simulink library "acc_control_lib"  (R2024a)
settings: Solver=VariableStepAuto  StartTime=0.0  StopTime=10.0  RelTol=1e-3
settings Model: Creator=26401  LastModifiedBy=26401

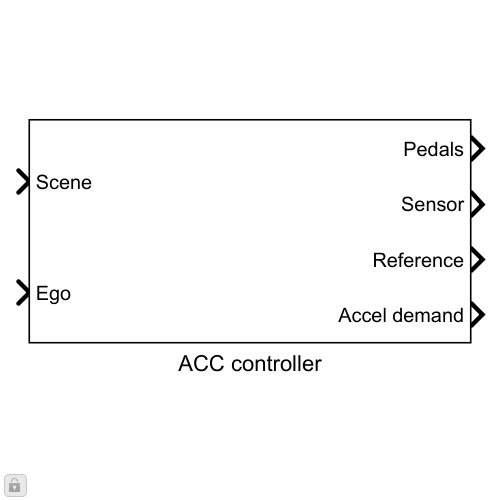
[thumbnail: Simulink's stored preview of the top-level diagram]
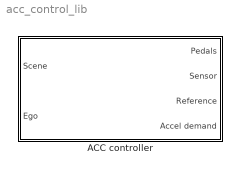
== system acc_control_lib ==
  ACC controller : Subsystem

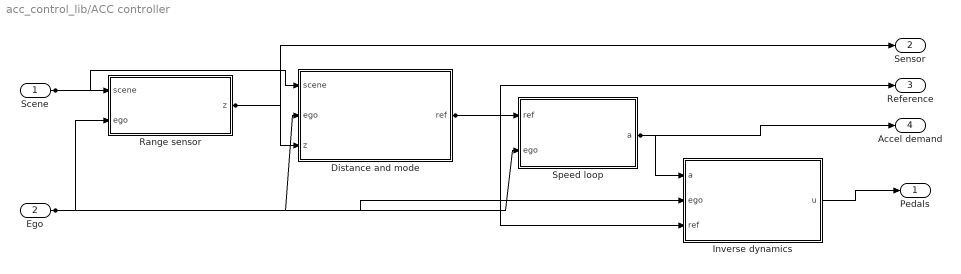
== system acc_control_lib/ACC controller ==
  Scene : Inport
  Ego : Inport  Port=2
  Distance and mode : MATLAB Function  TreatAsAtomicUnit=on
  Inverse dynamics : MATLAB Function  TreatAsAtomicUnit=on
  Range sensor : MATLAB Function  TreatAsAtomicUnit=on
  Speed loop : MATLAB Function  TreatAsAtomicUnit=on
  Pedals : Outport
  Sensor : Outport  Port=2
  Reference : Outport  Port=3
  Accel demand : Outport  Port=4
  wires:
  Scene/1 -> Range sensor/1(scene), Distance and mode/1(scene)
  Ego/1 -> Range sensor/2(ego), Distance and mode/2(ego), Speed loop/2(ego), Inverse dynamics/2(ego)
  Range sensor/1(z) -> Distance and mode/3(z), Sensor/1
  Distance and mode/1(ref) -> Speed loop/1(ref), Inverse dynamics/3(ref), Reference/1
  Speed loop/1(a) -> Inverse dynamics/1(a), Accel demand/1
  Inverse dynamics/1(u) -> Pedals/1

== matlab function acc_control_lib/ACC controller/Range sensor ==
  data: scene input; z output; ego input
function z = range_sensor(scene,ego)
% scene = [set speed, lead speed, lead rear s, target exists].
% ego = [front bumper s, speed, acceleration, engine rpm, transmission ratio].
% Negative gap remains visible for collision detection in a single-lane run.
gap = scene(3)-ego(1);
valid = scene(4)>0.5 && gap<=150;
z = [double(valid);0;0];
if valid
    z(2:3) = [gap;scene(2)-ego(2)];
end
end

== matlab function acc_control_lib/ACC controller/Speed loop ==
  data: ref input; a output; ego input
function a = speed_control(ref,ego)
% Inner P speed feedback, no integral accumulation across mode transitions.
% Local gains and slew limits. Requests refer to net longitudinal acceleration.
persistent previous
if isempty(previous)
    previous = 0;
end
demand = min(max(2.4*(ref(1)-ego(2)),-4),2.8);
if ref(4)>0.5
    demand = -1.0;
end
a = previous + min(max(demand-previous,-6*0.02),6*0.02);
previous = a;
end

== matlab function acc_control_lib/ACC controller/Inverse dynamics ==
  data: a input; u output; ego input; ref input
function u = inverse_actuators(a,ego,ref)
% Drive/brake hysteresis around the zero-pedal coasting acceleration.
% Throttle is normalized, master-cylinder pressure is in MPa.
persistent driving
if isempty(driving)
    driving = true;
end
[loss,fullForce,mass] = baseline_forces(ego(2),ego(4),ego(5));
coast = -loss/mass;
if a>coast+0.05
    driving = true;
elseif a<coast-0.05
    driving = false;
end
force = mass*(a-coast);
throttle = 0;
pressure = 0;
if driving
    throttle = min(max(force/fullForce,0),1);
else
    torque = max(-force*0.304,0);
    % Two front (350 N m/MPa) and two rear (200 N m/MPa) brakes.
    % Above 2 MPa the rear pressure slope falls to 0.3.
    if torque <= 2200
        pressure = torque/1100;
    else
        pressure = 2+(torque-2200)/820;
    end
    pressure = min(pressure,8);
end
if ref(4)>0.5
    throttle = 0; pressure = max(pressure,0.6); driving = false;
end
u = [throttle;pressure];
end

== matlab function acc_control_lib/ACC controller/Distance and mode ==
  data: scene input; ref output; ego input; z input
function ref = follow_reference(scene,ego,z)
% Output [speed request m/s, desired gap m, mode (1 ACC / 2 CC), hold].
% Filtered derivative of d - d0 - h*v, directly from the sensor and ego ax.
persistent following integral deriv hold
if isempty(following)
    following = false; integral = 0; deriv = 0; hold = false;
end
Ts = 0.02;
h = 3.6;
d0 = 5;
v = ego(2);
desiredGap = d0+h*v;
error = z(2)-desiredGap;
if ~logical(z(1))
    following = false;
elseif following
    if error>10 && z(3)>=0
        following = false;
    end
elseif error<=0
    following = true;
end
request = scene(1);
if z(1)>0.5
    deriv = deriv + Ts/(0.18+Ts)*(z(3)-h*ego(3)-deriv);
else
    deriv = 0;
end
if following
    correction = 0.8*error + integral + 0.3*deriv; % km/h
    dv = min(max(correction,-35),35);
    request = min(max(v+dv/3.6,0),scene(1));
    applied = (request-v)*3.6;
    integral = integral + Ts*(0.07*error + 0.035*(applied-correction));
    % Course stop-and-go latch. Release when the lead begins pulling away.
    leadSpeed = v+z(3);
    if hold
        hold = leadSpeed<0.5 && z(2)<d0+2;
    else
        hold = leadSpeed<0.10 && v<0.55 && z(2)<d0+0.8;
    end
    if hold
        request = 0; integral = 0; deriv = 0;
    end
else
    integral = 0; hold = false;
end
ref = [request;desiredGap;2-double(following);double(hold)];
end
